simulink model "MATE_SwitchedReluctanceMotor64Drive"  (R2024b)
settings: Solver=FixedStepDiscrete  StartTime=0.0  StopTime=5  FixedStep=Ts  RelTol=1e-3  AbsTol=1e-5  EnableMultiTasking=on
PreLoadFcn:
  | Ts=1e-6;Rsnu=100; Csnu=1e-6;
  | 
  | % Magnetisation characteristic table of the switched Reluctance Motor:
  | % Table elements =  Flux linkage, in Wb.
  | 
  | FluxTable = [
  |     0             0              0             0             0             0
  |     0.3220    0.3050    0.2280    0.1240    0.0220    0.0170
  |     0.3760    0.3570    0.2770    0.1600    0.0420    0.0340
  |     0.3990    0.3850    0.3000    0.1830    0.0640    0.0500
  |     0.4160    0.4020    0.3200    0.2010    0.0840    0.0670
  |     0.4280    0.4150    0.3340    0.2190    0.1030    0.0840
  |     0.4370    0.4260    0.3480    0.2370    0.1230    0.1010
  |     0.4430    0.4330    0.3590    0.2530    0.1420    0.1170
  |     0.4490    0.4390    0.3710    0.2680    0.1610    0.1340
  |     0.4540    0.4440    0.3820    0.2820    0.1790    0.1510
  |     0.4590    0.4490    0.3920    0.2950    0.1970    0.1680
  |     0.4630    0.4530    0.4020    0.3090    0.2140    0.1840
  |     0.4670    0.4570    0.4110    0.3220    0.2310    0.2010
  |     0.4700    0.4620    0.4190    0.3360    0.2460    0.2180
  |     0.4740    0.4650    0.4270    0.3480    0.2610    0.2350
  |     0.4780    0.4690    0.4330    0.3590    0.2770    0.2510
  |     0.4810    0.4730    0.4380    0.3690    0.2910    0.2680
  |     0.4840    0.4770    0.4440    0.3800    0.3050    0.2850
  |     0.4870    0.4790    0.4480    0.3890    0.3200    0.3020];
  | 
  | % Table columns :  Rotor angles, in degrees.
  | 
  | RotorAngles = [
  |     0             10            20            30            40            45];
  | 
  | % Table rows : Stator current, in A.
  | 
  | StatorCurrents = [ 0:size(FluxTable,1)-1] * 25;
PostLoadFcn:
  | Ts=1e-6;Rsnu=100; Csnu=1e-6;
  | 
  | % Magnetisation characteristic table of the switched Reluctance Motor:
  | % Table elements =  Flux linkage, in Wb.
  | 
  | FluxTable = [
  |     0             0              0             0             0             0
  |     0.3220    0.3050    0.2280    0.1240    0.0220    0.0170
  |     0.3760    0.3570    0.2770    0.1600    0.0420    0.0340
  |     0.3990    0.3850    0.3000    0.1830    0.0640    0.0500
  |     0.4160    0.4020    0.3200    0.2010    0.0840    0.0670
  |     0.4280    0.4150    0.3340    0.2190    0.1030    0.0840
  |     0.4370    0.4260    0.3480    0.2370    0.1230    0.1010
  |     0.4430    0.4330    0.3590    0.2530    0.1420    0.1170
  |     0.4490    0.4390    0.3710    0.2680    0.1610    0.1340
  |     0.4540    0.4440    0.3820    0.2820    0.1790    0.1510
  |     0.4590    0.4490    0.3920    0.2950    0.1970    0.1680
  |     0.4630    0.4530    0.4020    0.3090    0.2140    0.1840
  |     0.4670    0.4570    0.4110    0.3220    0.2310    0.2010
  |     0.4700    0.4620    0.4190    0.3360    0.2460    0.2180
  |     0.4740    0.4650    0.4270    0.3480    0.2610    0.2350
  |     0.4780    0.4690    0.4330    0.3590    0.2770    0.2510
  |     0.4810    0.4730    0.4380    0.3690    0.2910    0.2680
  |     0.4840    0.4770    0.4440    0.3800    0.3050    0.2850
  |     0.4870    0.4790    0.4480    0.3890    0.3200    0.3020];
  | 
  | % Table columns :  Rotor angles, in degrees.
  | 
  | RotorAngles = [
  |     0             10            20            30            40            45];
  | 
  | % Table rows : Stator current, in A.
  | 
  | StatorCurrents = [ 0:size(FluxTable,1)-1] * 25;
InitFcn:
  | Ts=1e-6;Rsnu=100; Csnu=1e-6;
  | 
  | % Magnetisation characteristic table of the switched Reluctance Motor:
  | % Table elements =  Flux linkage, in Wb.
  | 
  | FluxTable = [
  |     0             0              0             0             0             0
  |     0.3220    0.3050    0.2280    0.1240    0.0220    0.0170
  |     0.3760    0.3570    0.2770    0.1600    0.0420    0.0340
  |     0.3990    0.3850    0.3000    0.1830    0.0640    0.0500
  |     0.4160    0.4020    0.3200    0.2010    0.0840    0.0670
  |     0.4280    0.4150    0.3340    0.2190    0.1030    0.0840
  |     0.4370    0.4260    0.3480    0.2370    0.1230    0.1010
  |     0.4430    0.4330    0.3590    0.2530    0.1420    0.1170
  |     0.4490    0.4390    0.3710    0.2680    0.1610    0.1340
  |     0.4540    0.4440    0.3820    0.2820    0.1790    0.1510
  |     0.4590    0.4490    0.3920    0.2950    0.1970    0.1680
  |     0.4630    0.4530    0.4020    0.3090    0.2140    0.1840
  |     0.4670    0.4570    0.4110    0.3220    0.2310    0.2010
  |     0.4700    0.4620    0.4190    0.3360    0.2460    0.2180
  |     0.4740    0.4650    0.4270    0.3480    0.2610    0.2350
  |     0.4780    0.4690    0.4330    0.3590    0.2770    0.2510
  |     0.4810    0.4730    0.4380    0.3690    0.2910    0.2680
  |     0.4840    0.4770    0.4440    0.3800    0.3050    0.2850
  |     0.4870    0.4790    0.4480    0.3890    0.3200    0.3020];
  | 
  | % Table columns :  Rotor angles, in degrees.
  | 
  | RotorAngles = [
  |     0             10            20            30            40            45];
  | 
  | % Table rows : Stator current, in A.
  | 
  | StatorCurrents = [ 0:size(FluxTable,1)-1] * 25;
undefined symbols (not defined in the file or in its folder): DiscIntNeverNeededParam
libraries: ee_lib x12, nesl_utility x10, fl_lib x6, simetranss x5
(part 1 of 2)
Description:
  | Copyright 2008-2017 The MathWorks, Inc.
settings Model: ARTEMISmethode_block_infos=$$__separator__$$  ModifiedByFormat=Kyle  Creator=Kyle Diller  LastModifiedBy=Kyle
settings SolverCC: AutoScaleAbsTol=off  AlgebraicLoopSolver=TrustRegion  InsertRTBMode=Auto
settings DataIOCC: LimitDataPoints=on  SaveFormat=Array  SignalLoggingSaveFormat=ModelDataLogs  ReturnWorkspaceOutputs=off  SignalLoggingName=sigsOut
settings OptimizationCC: ExpressionDepthLimit=2147483647  InitFltsAndDblsToZero=on  LifeSpan=inf
settings DebuggingCC: UnderspecifiedInitializationDetection=Classic  MergeDetectMultiDrivingBlocksExec=none  CheckExecutionContextPreStartOutputMsg=on  SignalResolutionControl=TryResolveAllWithWarning  MultiTaskDSMMsg=warning  MultiTaskCondExecSysMsg=none  FcnCallInpInsideContextMsg=warning  UnconnectedInputMsg=warning  UnconnectedOutputMsg=warning  UnconnectedLineMsg=warning  StateNameClashWarn=warning  SFUnexpectedBacktrackingDiag=warning  SFNoUnconditionalDefaultTransitionDiag=warning  SFExecutionAtInitializationDiag=none  ArithmeticOperatorsInVariantConditions=warning
settings HardwareCC: ProdBitPerPointer=32  ProdBitPerSizeT=32  ProdBitPerPtrDiffT=32  ProdLargestAtomicFloat=None  ProdIntDivRoundTo=Undefined  ProdEndianess=Unspecified  ProdWordSize=32  ProdHWDeviceType=32-bit Generic  TargetUnknown=on
settings ModelReferenceCC: EnableRefExpFcnMdlSchedulingChecks=on  PropagateSignalLabelsOutOfModel=off
settings SFSimCC: SimUseLocalCustomCode=off  CustomCodeUndefinedFunction=UseInterfaceOnly
settings RTWCC: RTWUseLocalCustomCode=off  GPUComputeCapability=3.5
settings CodeAppCC: StateflowObjectComments=on
settings GRTTargetCC: TargetLangStandard=C89/C90 (ANSI)  CombineOutputUpdateFcns=off  GRTInterface=on
settings ConfigComp: CovMetricSettings=dw  CovSaveCumulativeToWorkspaceVar=on  CovSaveSingleToWorkspaceVar=on  CovExternalEMLEnable=off  CovSFcnEnable=off
settings SimscapeCC: SimscapeNormalizeSystem=off

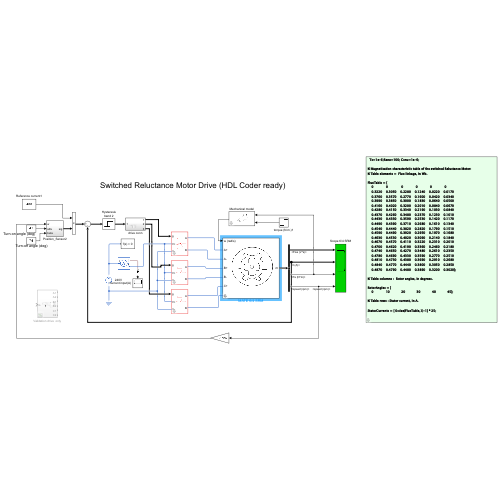
[thumbnail: Simulink's stored preview of the top-level diagram]
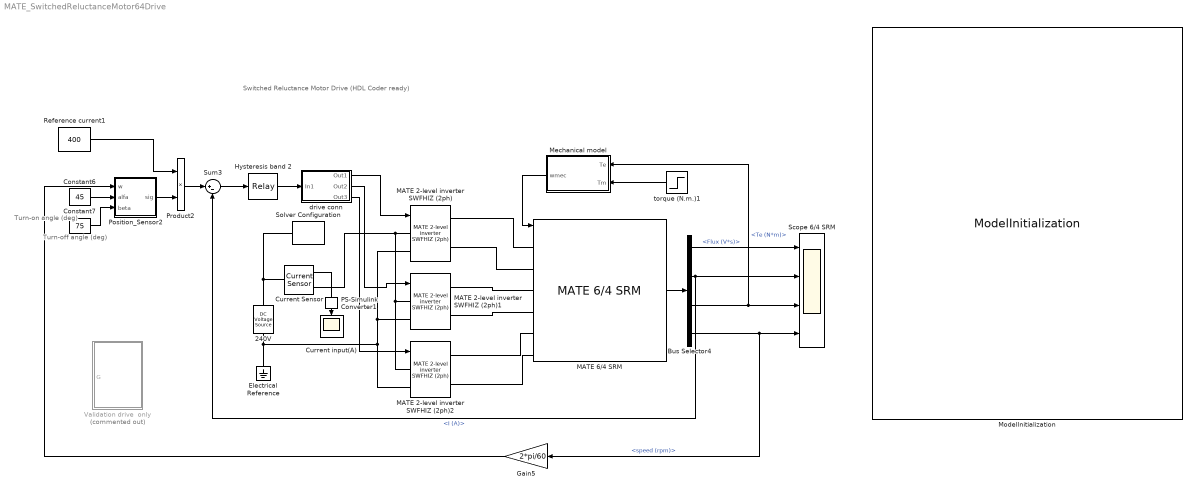
== system MATE_SwitchedReluctanceMotor64Drive ==
  note: Switched Reluctance Motor Drive (HDL Coder ready)
  note: Turn-off angle (deg)
  note: Turn-on angle (deg)
  240V : fl_lib/Electrical/Electrical Sources/DC Voltage Source  v0=240 V
  Bus Selector4 : BusSelector  OutputSignals=Flux (V*s),I (A),Te (N*m),speed (rpm)
  Constant6 : Constant  Value=45
  Constant7 : Constant  Value=75
  Current Sensor : fl_lib/Electrical/Electrical Sensors/Current Sensor
  Current input(A) : Scope
  Electrical Reference : fl_lib/Electrical/Electrical Elements/Electrical Reference
  Gain5 : Gain  Gain=2*pi/60  SaturateOnIntegerOverflow=on  OutDataTypeStr=Inherit: Same as input  ParamDataTypeStr=Inherit: Same as input
  Hysteresis band 2 : Relay  OnSwitchValue=10  OffSwitchValue=-10  SampleTime=Ts
  MATE 2-level inverter SWFHIZ (2ph) : simetranss/FPGA/MATE 2-level inverter SWFHIZ (2ph)  Ron=1e-3  Vf=0.8  Gpp=Rsnu  Gip=Csnu  Ts=Ts  min_charge=0.1
  MATE 2-level inverter SWFHIZ (2ph)1 : simetranss/FPGA/MATE 2-level inverter SWFHIZ (2ph)  Ron=1e-3  Vf=0.8  Gpp=Rsnu  Gip=Csnu  Ts=Ts  min_charge=0.1
  MATE 2-level inverter SWFHIZ (2ph)2 : simetranss/FPGA/MATE 2-level inverter SWFHIZ (2ph)  Ron=1e-3  Vf=0.8  Gpp=Rsnu  Gip=Csnu  Ts=Ts  min_charge=0.1
  MATE 6/4 SRM : simetranss/Machines/MATE 6//4 SRM  MachineType=6/4  Rs=0.05  Inertia=0.05  FluxTable=FluxTable  RotorAngles=RotorAngles  StatorCurrents=StatorCurrents  Friction=0.02  Initialangle=0  TsBlock=-1  nb_points=[100,20,20]  PlotCurves=on
  Mechanical model : Subsystem  mask(Machine rotational mechanical model){J=0.5, F=0.02, fo=0, Ts=Ts}
      mask prompts: J "Inertia (kg.m^2)"; F "Friction (N.m.s)"; fo "Initial mechanical frequency (Hz)"; Ts "Sample Time (s)"
      mask help:
      | This block can implement a simple rotating mechanical equation for machines
      |
      | The block working equation is:
      | wmec=1/J*INT{( Te - Tm -F*wmec )*dt}
      |
      | All values in SI.
      |
      | Parameters:
      | Inertia J (kg.m^2)
      | Friction F (N.m.s)
      | Initial mechanical frequency (Hz)
      | Sample Time (s).
      |
      | Signals:
      | Te: electric torque input from the machine (N.m.)
      | Tm : mechanical torque applied to the shaft (N.m.)
      | wmec: mechanical speed of machine (rad/s)
      |
      | Conversion from Per-Unit values
      |
      | J=2*H*Pn/w_mec^2
      | F=D*Pn/w_mec^2
      | where:
      | J is the inertia in km.m^2
      | H is the inertia constant in seconds.
      | F is the friction factor in N.m.s
      | D in the friction factor or damping factor in pu.
      | Pn is the nominal power of the machine
      | w_mec is the nominal mechanical rotational frequency of the machine in rad/s
  ModelInitialization : simetranss/Usefulls/ModelInitialization  InitFcnX=|  prel=on  posl=on  inif=on  strf=off
      | Ts=1e-6;Rsnu=100; Csnu=1e-6; 
      | 
      | % Magnetisation characteristic table of the switched Reluctance Motor:
      | % Table elements =  Flux linkage, in Wb.
      | 
      | FluxTable = [
      |     0             0              0             0             0             0
      |     0.3220    0.3050    0.2280    0.1240    0.0220    0.0170
      |     0.3760    0.3570    0.2770    0.1600    0.0420    0.0340
      |     0.3990    0.3850    0.3000    0.1830    0.0640    0.0500
      |     0.4160    0.4020    0.3200    0.2010    0.0840    0.0670
      |     0.4280    0.4150    0.3340    0.2190    0.1030    0.0840
      |     0.4370    0.4260    0.3480    0.2370    0.1230    0.1010
      |     0.4430    0.4330    0.3590    0.2530    0.1420    0.1170
      |     0.4490    0.4390    0.3710    0.2680    0.1610    0.1340
      |     0.4540    0.4440    0.3820    0.2820    0.1790    0.1510
      |     0.4590    0.4490    0.3920    0.2950    0.1970    0.1680
      |     0.4630    0.4530    0.4020    0.3090    0.2140    0.1840
      |     0.4670    0.4570    0.4110    0.3220    0.2310    0.2010
      |     0.4700    0.4620    0.4190    0.3360    0.2460    0.2180
      |     0.4740    0.4650    0.4270    0.3480    0.2610    0.2350
      |     0.4780    0.4690    0.4330    0.3590    0.2770    0.2510
      |     0.4810    0.4730    0.4380    0.3690    0.2910    0.2680
      |     0.4840    0.4770    0.4440    0.3800    0.3050    0.2850
      |     0.4870    0.4790    0.4480    0.3890    0.3200    0.3020]; 
      | 
      | % Table columns :  Rotor angles, in degrees.
      | 
      | RotorAngles = [
      |     0             10            20            30            40            45];
      | 
      | % Table rows : Stator current, in A.
      | 
      | StatorCurrents = [ 0:size(FluxTable,1)-1] * 25;
  PS-Simulink Converter1 : nesl_utility/PS-Simulink Converter  PhysicalDomain=network_engine_domain  SubClassName=ps_output  LeftPortType=input  RightPortType=output  PseudoPeriodic=off  Frequencies=[]  VectorFormat=inherit  Unit=inherit  AffineConversion=off
  Position_Sensor2 : Subsystem
  Product2 : Product  SaturateOnIntegerOverflow=on  OutDataTypeStr=Inherit: Same as first input
  Reference current1 : Constant  Value=400
  Scope 6/4 SRM : Scope  NumInputPorts=4
  Solver Configuration : nesl_utility/Solver Configuration  PhysicalDomain=network_engine_domain  SubClassName=solver  LeftPortType=input  RightPortType=generic  Tones=[]  Harmonics=[]  SimulateNoise=off  Profile=off  UseLocalSampling=off  EnableSwitchedLinearOptims=on  FrequencyDomain=off  UseCCode=off  RelTol=0.001  AbsTol=0.001  MinStep=1e-09  ToWorkspace=off  RevertToSquareIcSolve=off  NumHomotopyIterations=100  PhasorMode=off  PhasorModeNumHarmonics=1  ConsistencySolver=NEWTON_XTOL_AFTER_FTOL  IndexReductionMethod=DerivativeReplacement  DoDC=off  ResidualTolerance=1e-09  ConsistencyTolSource=GLOBAL  ConsistencyAbsTol=0.001  ConsistencyRelTol=0.001  ConsistencyTolFactor=0.001  UseLocalSolver=on  LocalSolverChoice=NE_BACKWARD_EULER_ADVANCER  ResolveIndetEquations=on  FunctionEvalNumThread=1  LocalSolverSampleTime=Ts  DoFixedCost=on  MaxNonlinIter=1  MaxModeIter=2  ComputeImpulses=off  ImpulseIterations=2  LinearAlgebra=auto  LinearAlgebraNumThread=0  EquationFormulation=NE_TIME_EF  DelaysMemoryBudget=1024  AutomaticFiltering=on  FilteringTimeConstant=0.001  PartitionStorageMethod=AS_NEEDED  PartitionMemoryBudget=1024  PartitionMethod=ROBUST  MultibodyUseLocalSolver=off  MultibodyLocalSolverChoice=ODE1  MultibodyLocalSolverSampleTime=0.001
  Sum3 : Sum  Inputs=|+-  SaturateOnIntegerOverflow=on
  Validation drive  only : Subsystem  Commented=on
  drive conn : Subsystem
  torque (N.m.)1 : Step  After=100  SampleTime=0
  wires:
  Bus Selector4/3 -> Mechanical model/1(Te), Scope 6/4 SRM/3  "<Te (N*m)>"
  Constant6/1 -> Position_Sensor2/2(alfa)
  Constant7/1 -> Position_Sensor2/3(beta)
  Sum3/1 -> Hysteresis band 2/1
  Product2/1 -> Sum3/1
  Position_Sensor2/1(sig) -> Product2/2
  MATE 6/4 SRM/1 -> Bus Selector4/1
  Bus Selector4/1 -> Scope 6/4 SRM/1  "<Flux (V*s)>"
  Bus Selector4/2 -> Scope 6/4 SRM/2, Sum3/2  "<I (A)>"
  Bus Selector4/4 -> Scope 6/4 SRM/4, Gain5/1  "<speed (rpm)>"
  torque (N.m.)1/1 -> Mechanical model/2(Tm)
  Gain5/1 -> Position_Sensor2/1(w)
  Mechanical model/1(wmec) -> MATE 6/4 SRM/1
  Reference current1/1 -> Product2/1
  PS-Simulink Converter1/1 -> Current input(A)/1
  Hysteresis band 2/1 -> drive conn/1(In1)
  drive conn/1(Out1) -> MATE 2-level inverter SWFHIZ (2ph)/1
  drive conn/2(Out2) -> MATE 2-level inverter SWFHIZ (2ph)1/1
  drive conn/3(Out3) -> MATE 2-level inverter SWFHIZ (2ph)2/1
  connections:
  Solver Configuration/RConn1 -- 240V/LConn1 -- Current Sensor/LConn1
  240V/RConn1 -- Electrical Reference/LConn1 -- MATE 2-level inverter SWFHIZ (2ph)1/LConn2 -- MATE 2-level inverter SWFHIZ (2ph)/LConn2 -- MATE 2-level inverter SWFHIZ (2ph)2/LConn2
  Current Sensor/RConn1 -- PS-Simulink Converter1/LConn1
  Current Sensor/RConn2 -- MATE 2-level inverter SWFHIZ (2ph)2/LConn1 -- MATE 2-level inverter SWFHIZ (2ph)1/LConn1 -- MATE 2-level inverter SWFHIZ (2ph)/LConn1
  MATE 2-level inverter SWFHIZ (2ph)/RConn1 -- MATE 6/4 SRM/LConn1
  MATE 2-level inverter SWFHIZ (2ph)1/RConn2 -- MATE 6/4 SRM/LConn4
  MATE 2-level inverter SWFHIZ (2ph)/RConn2 -- MATE 6/4 SRM/LConn2
  MATE 2-level inverter SWFHIZ (2ph)1/RConn1 -- MATE 6/4 SRM/LConn3
  MATE 2-level inverter SWFHIZ (2ph)2/RConn2 -- MATE 6/4 SRM/LConn6
  MATE 2-level inverter SWFHIZ (2ph)2/RConn1 -- MATE 6/4 SRM/LConn5

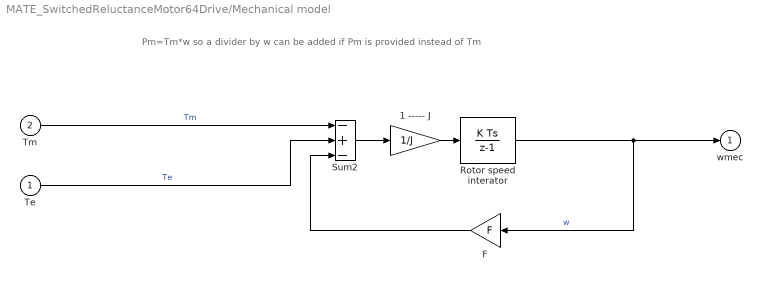
== system MATE_SwitchedReluctanceMotor64Drive/Mechanical model ==
  note: Pm=Tm*w so a divider by w can be added if Pm is provided instead of Tm
  Te : Inport  PortDimensions=1
  Tm : Inport  Port=2
  1 ----- J : Gain  Gain=1/J  SaturateOnIntegerOverflow=on  OutDataTypeStr=Inherit: Same as input  ParamDataTypeStr=Inherit: Same as input
  F : Gain  Gain=F  SaturateOnIntegerOverflow=on  OutDataTypeStr=Inherit: Same as input  ParamDataTypeStr=Inherit: Same as input
  Rotor speed interator : DiscreteIntegrator  InitialCondition=fo*2*pi  SampleTime=Ts  ICPrevOutput=DiscIntNeverNeededParam  ICPrevScaledInput=DiscIntNeverNeededParam
  Sum2 : Sum  Inputs=-+-  InputSameDT=on  SaturateOnIntegerOverflow=on  OutDataTypeStr=Inherit: Same as first input
  wmec : Outport  InitialOutput=0  VectorParamsAs1DForOutWhenUnconnected=off
  wires:
  Tm/1 -> Sum2/1  "Tm"
  Sum2/1 -> 1 ----- J/1
  F/1 -> Sum2/3
  Te/1 -> Sum2/2  "Te"
  1 ----- J/1 -> Rotor speed interator/1
  Rotor speed interator/1 -> wmec/1, F/1  "w"

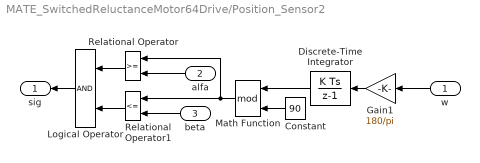
== system MATE_SwitchedReluctanceMotor64Drive/Position_Sensor2 ==
  w : Inport
  alfa : Inport  Port=2
  beta : Inport  Port=3
  Constant : Constant  Value=90
  Discrete-Time Integrator : DiscreteIntegrator  InitialCondition=[0 -30 -60]  SampleTime=Ts  ICPrevOutput=DiscIntNeverNeededParam  ICPrevScaledInput=DiscIntNeverNeededParam
  Gain1 : Gain  Gain=180/pi  SaturateOnIntegerOverflow=on  OutDataTypeStr=Inherit: Same as input  ParamDataTypeStr=Inherit: Same as input
  Logical Operator : Logic  AllPortsSameDT=off
  Math Function : Math  Operator=mod  SignedPower=on
  Relational Operator : RelationalOperator  InputSameDT=off
  Relational Operator1 : RelationalOperator  Operator=<=  InputSameDT=off
  sig : Outport  VectorParamsAs1DForOutWhenUnconnected=off
  wires:
  Logical Operator/1 -> sig/1
  w/1 -> Gain1/1
  Math Function/1 -> Relational Operator/1, Relational Operator1/1
  Relational Operator1/1 -> Logical Operator/2
  Gain1/1 -> Discrete-Time Integrator/1
  beta/1 -> Relational Operator1/2
  alfa/1 -> Relational Operator/2
  Relational Operator/1 -> Logical Operator/1
  Constant/1 -> Math Function/2
  Discrete-Time Integrator/1 -> Math Function/1

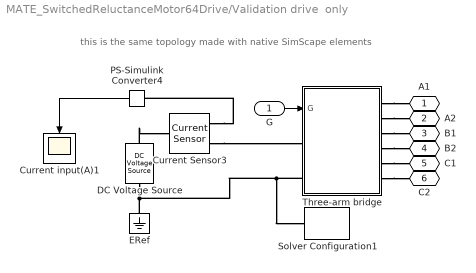
== system MATE_SwitchedReluctanceMotor64Drive/Validation drive  only ==
  note: this is the same topology made with native SimScape elements
  G : Inport
  Current Sensor3 : fl_lib/Electrical/Electrical Sensors/Current Sensor
  Current input(A)1 : Scope
  DC Voltage Source : fl_lib/Electrical/Electrical Sources/DC Voltage Source  v0=240 V
  ERef : fl_lib/Electrical/Electrical Elements/Electrical Reference
  PS-Simulink Converter4 : nesl_utility/PS-Simulink Converter  PhysicalDomain=network_engine_domain  SubClassName=ps_output  LeftPortType=input  RightPortType=output  PseudoPeriodic=off  Frequencies=[]  VectorFormat=inherit  Unit=inherit  AffineConversion=off
  Solver Configuration1 : nesl_utility/Solver Configuration  PhysicalDomain=network_engine_domain  SubClassName=solver  LeftPortType=input  RightPortType=generic  Tones=[]  Harmonics=[]  SimulateNoise=off  Profile=off  UseLocalSampling=off  EnableSwitchedLinearOptims=on  FrequencyDomain=off  UseCCode=off  RelTol=0.001  AbsTol=0.001  MinStep=1e-09  ToWorkspace=off  RevertToSquareIcSolve=off  NumHomotopyIterations=100  PhasorMode=off  PhasorModeNumHarmonics=1  ConsistencySolver=NEWTON_XTOL_AFTER_FTOL  IndexReductionMethod=DerivativeReplacement  DoDC=off  ResidualTolerance=1e-09  ConsistencyTolSource=GLOBAL  ConsistencyAbsTol=0.001  ConsistencyRelTol=0.001  ConsistencyTolFactor=0.001  UseLocalSolver=on  LocalSolverChoice=NE_BACKWARD_EULER_ADVANCER  ResolveIndetEquations=on  FunctionEvalNumThread=1  LocalSolverSampleTime=Ts  DoFixedCost=on  MaxNonlinIter=3  MaxModeIter=2  ComputeImpulses=off  ImpulseIterations=2  LinearAlgebra=auto  LinearAlgebraNumThread=0  EquationFormulation=NE_TIME_EF  DelaysMemoryBudget=1024  AutomaticFiltering=on  FilteringTimeConstant=0.001  PartitionStorageMethod=AS_NEEDED  PartitionMemoryBudget=1024  PartitionMethod=ROBUST  MultibodyUseLocalSolver=off  MultibodyLocalSolverChoice=ODE1  MultibodyLocalSolverSampleTime=0.001
  Three-arm bridge : Subsystem  Tag=PublishSubsystem
  A1 : PMIOPort  Side=Right
  A2 : PMIOPort  Port=2  Side=Right
  B1 : PMIOPort  Port=3  Side=Right
  B2 : PMIOPort  Port=4  Side=Right
  C1 : PMIOPort  Port=5  Side=Right
  C2 : PMIOPort  Port=6  Side=Right
  wires:
  PS-Simulink Converter4/1 -> Current input(A)1/1
  G/1 -> Three-arm bridge/1(G)
  connections:
  Three-arm bridge/LConn2 -- Solver Configuration1/RConn1 -- ERef/LConn1 -- DC Voltage Source/RConn1
  Current Sensor3/RConn2 -- Three-arm bridge/LConn1
  Three-arm bridge/RConn1 -- A1/RConn1
  Current Sensor3/RConn1 -- PS-Simulink Converter4/LConn1
  DC Voltage Source/LConn1 -- Current Sensor3/LConn1
  Three-arm bridge/RConn2 -- A2/RConn1
  Three-arm bridge/RConn3 -- B1/RConn1
  Three-arm bridge/RConn6 -- C2/RConn1
  Three-arm bridge/RConn4 -- B2/RConn1
  Three-arm bridge/RConn5 -- C1/RConn1

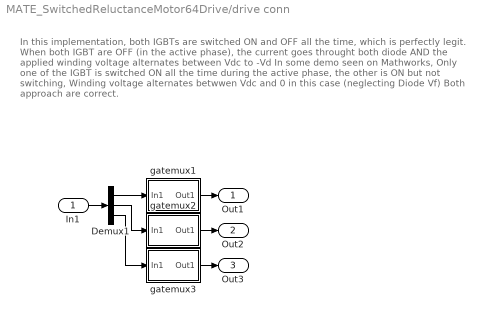
== system MATE_SwitchedReluctanceMotor64Drive/drive conn ==
  note: In this implementation, both IGBTs are switched ON and OFF all the time, which is perfectly legit. When both IGBT are OFF (in the active phase), the current goes throught both diode AND the applied winding voltage alternates between Vdc to -Vd
      |
      | In some demo seen on Mathworks, Only one of the IGBT is switched ON all the time during the active phase, the other is ON but not switching, Winding voltage alternates betwwen Vdc and 0 in this case (neglecting Diode Vf)
      |
      | Both approach are correct.
  In1 : Inport
  Demux1 : Demux  Outputs=3
  gatemux1 : Subsystem
  gatemux2 : Subsystem
  gatemux3 : Subsystem
  Out1 : Outport
  Out2 : Outport  Port=2
  Out3 : Outport  Port=3
  wires:
  Demux1/2 -> gatemux2/1(In1)
  gatemux1/1(Out1) -> Out1/1
  Demux1/1 -> gatemux1/1(In1)
  Demux1/3 -> gatemux3/1(In1)
  gatemux2/1(Out1) -> Out2/1
  gatemux3/1(Out1) -> Out3/1
  In1/1 -> Demux1/1

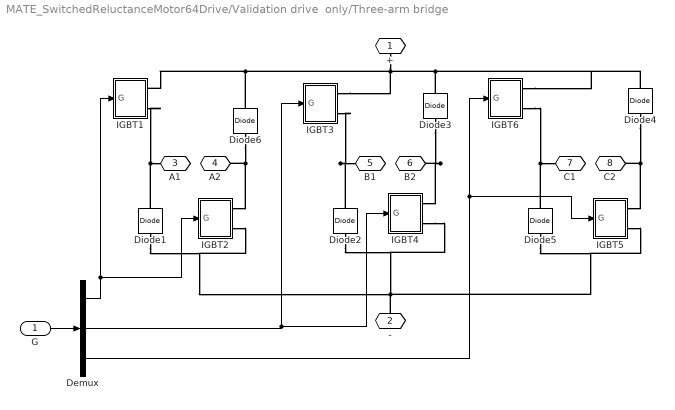
== system MATE_SwitchedReluctanceMotor64Drive/Validation drive  only/Three-arm bridge ==
  G : Inport
  Demux : Demux  Outputs=3
  Diode{1..6} (6 alike) : ee_lib/Semiconductors & Converters/Diode  ModelType=ee.enum.diode.modelType.pwl  TableType=ee.enum.diode.tableType.IfMat  IfMat=[.07, .12, .19, 1.75, 4.24, 7.32, 11.2; .16, .3, .72, 2.14, 5.02, 8.35, 13.12] A  VfMat=[.9, 1.15, 1.25, 1.5, 1.75, 2.17, 2.6, 2.85; .58, .68, .75, 1.1, 1.38, 1.77, 2.27, 2.7] V  TjVec=[25, 125] degC  VfVec=[.5, .7, .9, 1.3, 1.7, 2.1, 2.5] V  IfVec=[.1, .2, .5, 1, 2, 4, 7, 10] A  IrMat=[1e-06, 2e-06, 5e-06, 1e-05, 2.5e-05, 5e-05, .0001; 2e-06, 5e-06, 1e-05, 4e-05, 8e-05, .0002, .0005] A  VrMat=[10, 100, 200, 250, 300, 325, 350; 10, 70, 160, 220, 270, 300, 320] V  VrVec=[10, 20, 40, 50, 70, 80, 100] V  IrVec=[1e-06, 2e-06, 5e-06, 1e-05, 2e-05, 5e-05, .0001] A  Vf=0.1 V  Ron=0.01 Ohm  Goff=1e-8 1/Ohm  prmExp=ee.enum.diode.expParam.useTwo  I12=[.0137, .545] A  V12=[.6, .7] V  RS=0 Ohm  Tmeas=25 degC  IS=1e-12 A  ec=1  I1=0.0137 A  V1=0.6 V  N_series=1  N_parallel=1  ZenerEnable=false  Rz=0.3 Ohm  BV=inf V  C_param=ee.enum.diode.capParam.fixed  CJ=0 pF  CJ0=5 pF  Vvec=[.1, 10, 100] V  Cvec=[3.5, 1, .4] pF  VJ=1 V  Mgrad=0.5  FC=0.5  Q_param=ee.enum.diode.recoveryParam.off  iRM=-7.15 A  iF=4 A  didt=-750 A/us  trr_factor=3  trr=115 ns  Qrr=150 s*nA  Vr=-600 V  Ls=150 nH  Erec=0.03 J  TT=50 ns  tau=100 ns  T_param=ee.enum.diode.temperatureParam.off  Tdevice=25 degC  I1_T2=0.245 A  V1_T2=0.5 V  IS_T2=1.25e-7 A  Tmeas2=125 degC  XTI_param=ee.enum.diode.xtiParam.pn  XTI=3  EG_param=ee.enum.diode.egapParam.material_si  EG=1.11 eV  dBVdT=0 V/K  fault_action=simscape.enum.assert.action.none  t_fault=inf s  enable_fault_input=simscape.enum.onoff.off  i_specify=off  i_priority=None  i=0 A  i_nominal_specify=off  i_nominal_value=1  i_nominal_unit=A  v_specify=off  v_priority=None  v=0 V  v_nominal_specify=off  v_nominal_value=1  v_nominal_unit=V  v_capacitor_specify=off  v_capacitor_priority=None  v_capacitor=0 V  v_capacitor_nominal_specify=off  v_capacitor_nominal_value=1  v_capacitor_nominal_unit=V  Qj_specify=off  Qj_priority=High  Qj=0 C  Qj_nominal_specify=off  Qj_nominal_value=1  Qj_nominal_unit=C  i_diode_specify=off  i_diode_priority=None  i_diode=0 A  i_diode_nominal_specify=off  i_diode_nominal_value=1  i_diode_nominal_unit=A  v_diode_specify=off  v_diode_priority=None  v_diode=0 V  v_diode_nominal_specify=off  v_diode_nominal_value=1  v_diode_nominal_unit=V  i_capacitor_specify=off  i_capacitor_priority=None  i_capacitor=0 A  i_capacitor_nominal_specify=off  i_capacitor_nominal_value=1  i_capacitor_nominal_unit=A  power_dissipated_specify=off  power_dissipated_priority=None  power_dissipated=0 W  power_dissipated_nominal_specify=off  power_dissipated_nominal_value=1  power_dissipated_nominal_unit=W  fidelity_level=ee.enum.diode.fidelity.includeChargeDyn  rec_loss_model=ee.enum.diode.reverseRecoveryModel.fixed  ErecVal=0 J  scaleWithIandV=true  ErecMat=zeros(2, 3) J  TjrecVec=[298.15, 398.15] K  IfrecVec=[.1, 1, 10] A  IrecVal=10 A  VrecVal=10 V  tFilter=1 / 1000 / 100 s  thermal_network_parameterization=ee.enum.thermalNetworkTopology.junctionCase  Rth=[0, 10] K/W  Rth_Cauer=[1, 3, 10] K/W  Rth_Foster=[4, 6] K/W  thermal_mass_parameterization=ee.enum.thermalNetwork.timeconstant  thermal_mass=[0, 1] J/K  thermal_mass_Cauer=[.1, .3, 1] J/K  thermal_mass_Foster=[1.5, 3] J/K  thermal_time_constant=[0, 10] s  thermal_time_constant_Cauer=[1, 3, 10] s  thermal_time_constant_Foster=[6, 18] s  thermal_mass_initial_temperatures=[25, 25] degC  thermal_mass_initial_temperatures_Cauer=[25, 25, 25] degC  junction_thermal_mass=0.01 J/K  Tvec_initial_Foster=[25, 25, 25, 25] degC  no_thermal_network=0  junction_temperature_specify=off  junction_temperature_priority=None  junction_temperature=25 degC  junction_temperature_nominal_specify=off  junction_temperature_nominal_value=1  junction_temperature_nominal_unit=degC
  IGBT1 : Subsystem
  IGBT2 : Subsystem
  IGBT3 : Subsystem
  IGBT4 : Subsystem
  IGBT5 : Subsystem
  IGBT6 : Subsystem
  + : PMIOPort  Side=Left
  - : PMIOPort  Port=2  Side=Left
  A1 : PMIOPort  Port=3  Side=Right
  A2 : PMIOPort  Port=4  Side=Right
  B1 : PMIOPort  Port=5  Side=Right
  B2 : PMIOPort  Port=6  Side=Right
  C1 : PMIOPort  Port=7  Side=Right
  C2 : PMIOPort  Port=8  Side=Right
  wires:
  Demux/1 -> IGBT2/1(G), IGBT1/1(G)
  G/1 -> Demux/1
  Demux/2 -> IGBT4/1(G), IGBT3/1(G)
  Demux/3 -> IGBT5/1(G), IGBT6/1(G)
  connections:
  IGBT1/RConn2 -- A1/RConn1 -- Diode1/RConn1
  IGBT4/RConn2 -- Diode2/LConn1 -- -/RConn1 -- IGBT2/RConn2 -- Diode1/LConn1 -- IGBT5/RConn2 -- Diode5/LConn1
  Diode3/RConn1 -- IGBT6/RConn1 -- Diode4/RConn1 -- IGBT3/RConn1 -- Diode6/RConn1 -- IGBT1/RConn1 -- +/RConn1
  C1/RConn1 -- IGBT6/RConn2 -- Diode5/RConn1
  B1/RConn1 -- IGBT3/RConn2 -- Diode2/RConn1
  A2/RConn1 -- IGBT2/RConn1 -- Diode6/LConn1
  B2/RConn1 -- IGBT4/RConn1 -- Diode3/LConn1
  C2/RConn1 -- IGBT5/RConn1 -- Diode4/LConn1

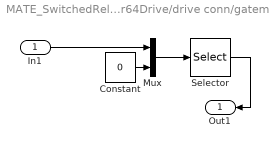
== system MATE_SwitchedReluctanceMotor64Drive/drive conn/gatemux1 ==
  In1 : Inport
  Constant : Constant  Value=0
  Mux : Mux  Inputs=2
  Selector : Selector  InputPortWidth=2  IndexOptions=Index vector (dialog)  Indices=[1 2 2 1]  OutputSizes=1
  Out1 : Outport
  wires:
  Selector/1 -> Out1/1
  In1/1 -> Mux/1
  Mux/1 -> Selector/1
  Constant/1 -> Mux/2

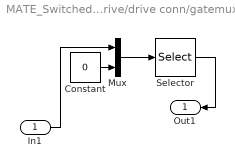
== system MATE_SwitchedReluctanceMotor64Drive/drive conn/gatemux2 ==
  In1 : Inport
  Constant : Constant  Value=0
  Mux : Mux  Inputs=2
  Selector : Selector  InputPortWidth=2  IndexOptions=Index vector (dialog)  Indices=[1 2 2 1]  OutputSizes=1
  Out1 : Outport
  wires:
  Constant/1 -> Mux/2
  Mux/1 -> Selector/1
  In1/1 -> Mux/1
  Selector/1 -> Out1/1

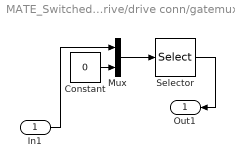
== system MATE_SwitchedReluctanceMotor64Drive/drive conn/gatemux3 ==
  In1 : Inport
  Constant : Constant  Value=0
  Mux : Mux  Inputs=2
  Selector : Selector  InputPortWidth=2  IndexOptions=Index vector (dialog)  Indices=[1 2 2 1]  OutputSizes=1
  Out1 : Outport
  wires:
  Selector/1 -> Out1/1
  In1/1 -> Mux/1
  Mux/1 -> Selector/1
  Constant/1 -> Mux/2

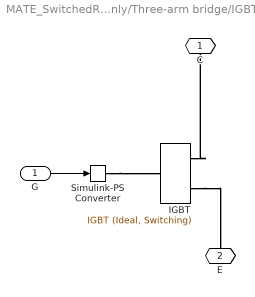
== system MATE_SwitchedReluctanceMotor64Drive/Validation drive  only/Three-arm bridge/IGBT1 ==
  G : Inport
  IGBT : ee_lib/Semiconductors & Converters/IGBT (Ideal, Switching)  port_option=ee.enum.controlport.ps  Vf=0.1 V  Ron=0.01 Ohm  Goff=1e-5 1/Ohm  Vth=0.5 V  diode_param=ee.enum.semiconductors.protectionDiode.external  diode_Vf=0.6 V  diode_Ron=0.03 Ohm  diode_Goff=1e-5 1/Ohm  diode_C=5e-8 F  diode_iRM=-235 A  diode_iF=300 A  diode_idot=-50 A/us  diode_trr_param=1  diode_trr_factor=3  diode_trr=15 us  diode_Qrr=1.5e+3 s*uA  ice_specify=off  ice_priority=None  ice=0 A  ice_nominal_specify=off  ice_nominal_value=1  ice_nominal_unit=A  vce_specify=off  vce_priority=None  vce=0 V  vce_nominal_specify=off  vce_nominal_value=1  vce_nominal_unit=V  vge_specify=off  vge_priority=None  vge=0 V  vge_nominal_specify=off  vge_nominal_value=1  vge_nominal_unit=V  thermal_loss_option=ee.enum.converters.thermalLossOption.constantvalues  Von_data=[0, .1, .6, .8, 1, 1.3, 1.6, 2, 2.4; 0, .1, .7, 1, 1.2, 1.5, 1.9, 2.4, 2.8] V  Tj=[298.15, 398.15] K  Iout_data=[0, .1, 1, 5, 10, 20, 40, 70, 100] A  Eon_data=[0, .0024, .024, .12, .2, .48, 1.04, 2.16, 3.24; 0, .003, .03, .15, .25, .6, 1.3, 2.7, 4.05] * 1e-3 J  Eoff_data=[0, .0007, .0066, .033, .066, .17, .33, .83, 1.5; 0, .001, .01, .05, .1, .25, .5, 1.2, 2.2] * 1e-3 J  Eon_data_3D=[zeros(2, 9, 3)] J  Eoff_data_3D=[zeros(2, 9, 3)] J  Tj_loss=[298.15, 398.15] K  Iout_data_loss=[0, .1, 1, 5, 10, 20, 40, 70, 100] A  tabulateWithVce=false  Vce_loss=[0, 150, 300] V  Eon_scalar=22.86e-3 J  Eoff_scalar=17.14e-3 J  Voff=300 V  Iout_scalar=600 A  useCurrentFromPreviousCycle=false  useVoltageFromPreviousCycle=false  diodeModelType=ee.enum.converters.diodeModelType.pwl  diodeTableType=ee.enum.diode.tableType.IfMat  diode_ReverseIVType=ee.enum.diode.diodeReverseIV.constant  diode_IfMat=[.07, .12, .19, 1.75, 4.24, 7.32, 11.2; .16, .3, .72, 2.14, 4.02, 6.35, 9.12] A  diode_VfMat=[.9, 1.15, 1.25, 1.5, 1.75, 2.17, 2.6, 2.85; .58, .68, .75, 1.1, 1.38, 1.77, 2.27, 2.7] V  diode_TjVec=[25, 125] degC  diode_VfVec=[.5, .7, .9, 1.3, 1.7, 2.1, 2.5] V  diode_IfVec=[.1, .2, .5, 1, 2, 4, 7, 10] A  diode_IrMat=[1e-06, 2e-06, 5e-06, 1e-05, 2.5e-05, 5e-05, .0001; 2e-06, 5e-06, 1e-05, 4e-05, 8e-05, .0002, .0005] A  diode_VrMat=[10, 100, 200, 250, 300, 325, 350; 10, 70, 160, 220, 270, 300, 320] V  diode_VrVec=[10, 20, 40, 50, 70, 80, 100] V  diode_IrVec=[1e-06, 2e-06, 5e-06, 1e-05, 2e-05, 5e-05, .0001] A  diode_Vr=-600 V  diode_Ls=150 nH  diode_Erec=0.03 J  diode_rec_loss_model=ee.enum.diode.reverseRecoveryModel.fixed  diode_ErecVal=0 J  diode_scaleWithIandV=true  diode_ErecMat=zeros(2, 3) J  diode_TjrecVec=[298.15, 398.15] K  diode_IfrecVec=[.1, 1, 10] A  diode_IrecVal=10 A  diode_VrecVal=10 V  diode_tFilter=1 / 1000 / 100 s  separateThermalPortForDiode=false  thermal_network_parameterization=ee.enum.thermalNetworkTopology.external  Rth=[.08, .5] K/W  Rth_Cauer=[.08, .1, .5] K/W  Rth_Foster=[.08, .14, .22, .16] K/W  thermal_mass_parameterization=ee.enum.thermalNetwork.timeconstant  thermal_mass=[.01, .5] J/K  thermal_mass_Cauer=[.01, .1, .5] J/K  thermal_mass_Foster=[.001, .005, .05, .5] J/K  thermal_time_constant=[.001, .2] s  thermal_time_constant_Cauer=[.001, .1, .2] s  thermal_time_constant_Foster=[7e-05, .0007, .01, .08] s  thermal_mass_initial_temperatures=[25, 25] degC  thermal_mass_initial_temperatures_Cauer=[25, 25, 25] degC  junction_thermal_mass=0.01 J/K  Tvec_initial_Foster=[25, 25, 25, 25] degC  RthDiode=[.03, .2] K/W  RthCauerDiode=[.03, .1, .2] K/W  RthFosterDiode=[.03, .2] K/W  thermalMassDiode=[3, 25] J/K  thermalMassCauerDiode=[3, 10, 25] J/K  thermalMassFosterDiode=[33, 50] J/K  thermalTauDiode=[.1, 5] s  thermalTauCauerDiode=[.1, 1, 5] s  thermalTauFosterDiode=[1, 10] s  thermalMassInitTempDiode=[25, 25] degC  thermalMassInitTempCauerDiode=[25, 25, 25] degC  junctionthermalMassDiode=0.1 J/K  TVecInitialFosterDiode=[25, 25, 25, 25] degC  no_thermal_network=0  IGBT_junction_temperature_specify=off  IGBT_junction_temperature_priority=None  IGBT_junction_temperature=25 degC  IGBT_junction_temperature_nominal_specify=off  IGBT_junction_temperature_nominal_value=1  IGBT_junction_temperature_nominal_unit=degC  diode_junction_temperature_specify=off  diode_junction_temperature_priority=None  diode_junction_temperature=25 degC  diode_junction_temperature_nominal_specify=off  diode_junction_temperature_nominal_value=1  diode_junction_temperature_nominal_unit=degC  Qj_specify=off  Qj_priority=None  Qj=0 W  Qj_nominal_specify=off  Qj_nominal_value=1  Qj_nominal_unit=W  accumulatedSwitchingLosses_specify=off  accumulatedSwitchingLosses_priority=None  accumulatedSwitchingLosses=0 J
  Simulink-PS Converter : nesl_utility/Simulink-PS Converter  PhysicalDomain=network_engine_domain  SubClassName=ps_input  LeftPortType=input  RightPortType=output  PseudoPeriodic=off  Frequencies=[]  NoiseDistribution=none  NoiseParameters=[]  Unit=V  AffineConversion=off  FilteringAndDerivatives=zero  SimscapeFilterOrder=1  InputFilterTimeConstant=.001  UdotUserProvided=1
  C : PMIOPort  Side=Right
  E : PMIOPort  Port=2  Side=Right
  wires:
  G/1 -> Simulink-PS Converter/1
  connections:
  IGBT/RConn1 -- C/RConn1
  IGBT/RConn2 -- E/RConn1
  Simulink-PS Converter/RConn1 -- IGBT/LConn1

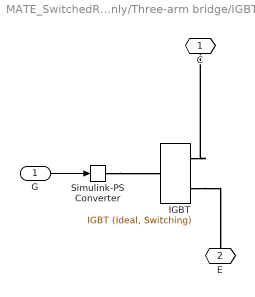
== system MATE_SwitchedReluctanceMotor64Drive/Validation drive  only/Three-arm bridge/IGBT2 ==
  G : Inport
  IGBT : ee_lib/Semiconductors & Converters/IGBT (Ideal, Switching)  port_option=ee.enum.controlport.ps  Vf=0.1 V  Ron=0.01 Ohm  Goff=1e-5 1/Ohm  Vth=0.5 V  diode_param=ee.enum.semiconductors.protectionDiode.external  diode_Vf=0.6 V  diode_Ron=0.03 Ohm  diode_Goff=1e-5 1/Ohm  diode_C=5e-8 F  diode_iRM=-235 A  diode_iF=300 A  diode_idot=-50 A/us  diode_trr_param=1  diode_trr_factor=3  diode_trr=15 us  diode_Qrr=1.5e+3 s*uA  ice_specify=off  ice_priority=None  ice=0 A  ice_nominal_specify=off  ice_nominal_value=1  ice_nominal_unit=A  vce_specify=off  vce_priority=None  vce=0 V  vce_nominal_specify=off  vce_nominal_value=1  vce_nominal_unit=V  vge_specify=off  vge_priority=None  vge=0 V  vge_nominal_specify=off  vge_nominal_value=1  vge_nominal_unit=V  thermal_loss_option=ee.enum.converters.thermalLossOption.constantvalues  Von_data=[0, .1, .6, .8, 1, 1.3, 1.6, 2, 2.4; 0, .1, .7, 1, 1.2, 1.5, 1.9, 2.4, 2.8] V  Tj=[298.15, 398.15] K  Iout_data=[0, .1, 1, 5, 10, 20, 40, 70, 100] A  Eon_data=[0, .0024, .024, .12, .2, .48, 1.04, 2.16, 3.24; 0, .003, .03, .15, .25, .6, 1.3, 2.7, 4.05] * 1e-3 J  Eoff_data=[0, .0007, .0066, .033, .066, .17, .33, .83, 1.5; 0, .001, .01, .05, .1, .25, .5, 1.2, 2.2] * 1e-3 J  Eon_data_3D=[zeros(2, 9, 3)] J  Eoff_data_3D=[zeros(2, 9, 3)] J  Tj_loss=[298.15, 398.15] K  Iout_data_loss=[0, .1, 1, 5, 10, 20, 40, 70, 100] A  tabulateWithVce=false  Vce_loss=[0, 150, 300] V  Eon_scalar=22.86e-3 J  Eoff_scalar=17.14e-3 J  Voff=300 V  Iout_scalar=600 A  useCurrentFromPreviousCycle=false  useVoltageFromPreviousCycle=false  diodeModelType=ee.enum.converters.diodeModelType.pwl  diodeTableType=ee.enum.diode.tableType.IfMat  diode_ReverseIVType=ee.enum.diode.diodeReverseIV.constant  diode_IfMat=[.07, .12, .19, 1.75, 4.24, 7.32, 11.2; .16, .3, .72, 2.14, 4.02, 6.35, 9.12] A  diode_VfMat=[.9, 1.15, 1.25, 1.5, 1.75, 2.17, 2.6, 2.85; .58, .68, .75, 1.1, 1.38, 1.77, 2.27, 2.7] V  diode_TjVec=[25, 125] degC  diode_VfVec=[.5, .7, .9, 1.3, 1.7, 2.1, 2.5] V  diode_IfVec=[.1, .2, .5, 1, 2, 4, 7, 10] A  diode_IrMat=[1e-06, 2e-06, 5e-06, 1e-05, 2.5e-05, 5e-05, .0001; 2e-06, 5e-06, 1e-05, 4e-05, 8e-05, .0002, .0005] A  diode_VrMat=[10, 100, 200, 250, 300, 325, 350; 10, 70, 160, 220, 270, 300, 320] V  diode_VrVec=[10, 20, 40, 50, 70, 80, 100] V  diode_IrVec=[1e-06, 2e-06, 5e-06, 1e-05, 2e-05, 5e-05, .0001] A  diode_Vr=-600 V  diode_Ls=150 nH  diode_Erec=0.03 J  diode_rec_loss_model=ee.enum.diode.reverseRecoveryModel.fixed  diode_ErecVal=0 J  diode_scaleWithIandV=true  diode_ErecMat=zeros(2, 3) J  diode_TjrecVec=[298.15, 398.15] K  diode_IfrecVec=[.1, 1, 10] A  diode_IrecVal=10 A  diode_VrecVal=10 V  diode_tFilter=1 / 1000 / 100 s  separateThermalPortForDiode=false  thermal_network_parameterization=ee.enum.thermalNetworkTopology.external  Rth=[.08, .5] K/W  Rth_Cauer=[.08, .1, .5] K/W  Rth_Foster=[.08, .14, .22, .16] K/W  thermal_mass_parameterization=ee.enum.thermalNetwork.timeconstant  thermal_mass=[.01, .5] J/K  thermal_mass_Cauer=[.01, .1, .5] J/K  thermal_mass_Foster=[.001, .005, .05, .5] J/K  thermal_time_constant=[.001, .2] s  thermal_time_constant_Cauer=[.001, .1, .2] s  thermal_time_constant_Foster=[7e-05, .0007, .01, .08] s  thermal_mass_initial_temperatures=[25, 25] degC  thermal_mass_initial_temperatures_Cauer=[25, 25, 25] degC  junction_thermal_mass=0.01 J/K  Tvec_initial_Foster=[25, 25, 25, 25] degC  RthDiode=[.03, .2] K/W  RthCauerDiode=[.03, .1, .2] K/W  RthFosterDiode=[.03, .2] K/W  thermalMassDiode=[3, 25] J/K  thermalMassCauerDiode=[3, 10, 25] J/K  thermalMassFosterDiode=[33, 50] J/K  thermalTauDiode=[.1, 5] s  thermalTauCauerDiode=[.1, 1, 5] s  thermalTauFosterDiode=[1, 10] s  thermalMassInitTempDiode=[25, 25] degC  thermalMassInitTempCauerDiode=[25, 25, 25] degC  junctionthermalMassDiode=0.1 J/K  TVecInitialFosterDiode=[25, 25, 25, 25] degC  no_thermal_network=0  IGBT_junction_temperature_specify=off  IGBT_junction_temperature_priority=None  IGBT_junction_temperature=25 degC  IGBT_junction_temperature_nominal_specify=off  IGBT_junction_temperature_nominal_value=1  IGBT_junction_temperature_nominal_unit=degC  diode_junction_temperature_specify=off  diode_junction_temperature_priority=None  diode_junction_temperature=25 degC  diode_junction_temperature_nominal_specify=off  diode_junction_temperature_nominal_value=1  diode_junction_temperature_nominal_unit=degC  Qj_specify=off  Qj_priority=None  Qj=0 W  Qj_nominal_specify=off  Qj_nominal_value=1  Qj_nominal_unit=W  accumulatedSwitchingLosses_specify=off  accumulatedSwitchingLosses_priority=None  accumulatedSwitchingLosses=0 J
  Simulink-PS Converter : nesl_utility/Simulink-PS Converter  PhysicalDomain=network_engine_domain  SubClassName=ps_input  LeftPortType=input  RightPortType=output  PseudoPeriodic=off  Frequencies=[]  NoiseDistribution=none  NoiseParameters=[]  Unit=V  AffineConversion=off  FilteringAndDerivatives=zero  SimscapeFilterOrder=1  InputFilterTimeConstant=.001  UdotUserProvided=1
  C : PMIOPort  Side=Right
  E : PMIOPort  Port=2  Side=Right
  wires:
  G/1 -> Simulink-PS Converter/1
  connections:
  Simulink-PS Converter/RConn1 -- IGBT/LConn1
  IGBT/RConn2 -- E/RConn1
  IGBT/RConn1 -- C/RConn1

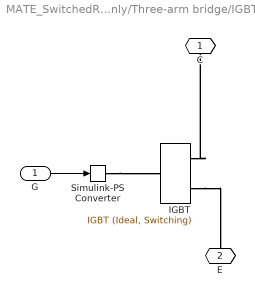
== system MATE_SwitchedReluctanceMotor64Drive/Validation drive  only/Three-arm bridge/IGBT3 ==
  G : Inport
  IGBT : ee_lib/Semiconductors & Converters/IGBT (Ideal, Switching)  port_option=ee.enum.controlport.ps  Vf=0.1 V  Ron=0.01 Ohm  Goff=1e-5 1/Ohm  Vth=0.5 V  diode_param=ee.enum.semiconductors.protectionDiode.external  diode_Vf=0.6 V  diode_Ron=0.03 Ohm  diode_Goff=1e-5 1/Ohm  diode_C=5e-8 F  diode_iRM=-235 A  diode_iF=300 A  diode_idot=-50 A/us  diode_trr_param=1  diode_trr_factor=3  diode_trr=15 us  diode_Qrr=1.5e+3 s*uA  ice_specify=off  ice_priority=None  ice=0 A  ice_nominal_specify=off  ice_nominal_value=1  ice_nominal_unit=A  vce_specify=off  vce_priority=None  vce=0 V  vce_nominal_specify=off  vce_nominal_value=1  vce_nominal_unit=V  vge_specify=off  vge_priority=None  vge=0 V  vge_nominal_specify=off  vge_nominal_value=1  vge_nominal_unit=V  thermal_loss_option=ee.enum.converters.thermalLossOption.constantvalues  Von_data=[0, .1, .6, .8, 1, 1.3, 1.6, 2, 2.4; 0, .1, .7, 1, 1.2, 1.5, 1.9, 2.4, 2.8] V  Tj=[298.15, 398.15] K  Iout_data=[0, .1, 1, 5, 10, 20, 40, 70, 100] A  Eon_data=[0, .0024, .024, .12, .2, .48, 1.04, 2.16, 3.24; 0, .003, .03, .15, .25, .6, 1.3, 2.7, 4.05] * 1e-3 J  Eoff_data=[0, .0007, .0066, .033, .066, .17, .33, .83, 1.5; 0, .001, .01, .05, .1, .25, .5, 1.2, 2.2] * 1e-3 J  Eon_data_3D=[zeros(2, 9, 3)] J  Eoff_data_3D=[zeros(2, 9, 3)] J  Tj_loss=[298.15, 398.15] K  Iout_data_loss=[0, .1, 1, 5, 10, 20, 40, 70, 100] A  tabulateWithVce=false  Vce_loss=[0, 150, 300] V  Eon_scalar=22.86e-3 J  Eoff_scalar=17.14e-3 J  Voff=300 V  Iout_scalar=600 A  useCurrentFromPreviousCycle=false  useVoltageFromPreviousCycle=false  diodeModelType=ee.enum.converters.diodeModelType.pwl  diodeTableType=ee.enum.diode.tableType.IfMat  diode_ReverseIVType=ee.enum.diode.diodeReverseIV.constant  diode_IfMat=[.07, .12, .19, 1.75, 4.24, 7.32, 11.2; .16, .3, .72, 2.14, 4.02, 6.35, 9.12] A  diode_VfMat=[.9, 1.15, 1.25, 1.5, 1.75, 2.17, 2.6, 2.85; .58, .68, .75, 1.1, 1.38, 1.77, 2.27, 2.7] V  diode_TjVec=[25, 125] degC  diode_VfVec=[.5, .7, .9, 1.3, 1.7, 2.1, 2.5] V  diode_IfVec=[.1, .2, .5, 1, 2, 4, 7, 10] A  diode_IrMat=[1e-06, 2e-06, 5e-06, 1e-05, 2.5e-05, 5e-05, .0001; 2e-06, 5e-06, 1e-05, 4e-05, 8e-05, .0002, .0005] A  diode_VrMat=[10, 100, 200, 250, 300, 325, 350; 10, 70, 160, 220, 270, 300, 320] V  diode_VrVec=[10, 20, 40, 50, 70, 80, 100] V  diode_IrVec=[1e-06, 2e-06, 5e-06, 1e-05, 2e-05, 5e-05, .0001] A  diode_Vr=-600 V  diode_Ls=150 nH  diode_Erec=0.03 J  diode_rec_loss_model=ee.enum.diode.reverseRecoveryModel.fixed  diode_ErecVal=0 J  diode_scaleWithIandV=true  diode_ErecMat=zeros(2, 3) J  diode_TjrecVec=[298.15, 398.15] K  diode_IfrecVec=[.1, 1, 10] A  diode_IrecVal=10 A  diode_VrecVal=10 V  diode_tFilter=1 / 1000 / 100 s  separateThermalPortForDiode=false  thermal_network_parameterization=ee.enum.thermalNetworkTopology.external  Rth=[.08, .5] K/W  Rth_Cauer=[.08, .1, .5] K/W  Rth_Foster=[.08, .14, .22, .16] K/W  thermal_mass_parameterization=ee.enum.thermalNetwork.timeconstant  thermal_mass=[.01, .5] J/K  thermal_mass_Cauer=[.01, .1, .5] J/K  thermal_mass_Foster=[.001, .005, .05, .5] J/K  thermal_time_constant=[.001, .2] s  thermal_time_constant_Cauer=[.001, .1, .2] s  thermal_time_constant_Foster=[7e-05, .0007, .01, .08] s  thermal_mass_initial_temperatures=[25, 25] degC  thermal_mass_initial_temperatures_Cauer=[25, 25, 25] degC  junction_thermal_mass=0.01 J/K  Tvec_initial_Foster=[25, 25, 25, 25] degC  RthDiode=[.03, .2] K/W  RthCauerDiode=[.03, .1, .2] K/W  RthFosterDiode=[.03, .2] K/W  thermalMassDiode=[3, 25] J/K  thermalMassCauerDiode=[3, 10, 25] J/K  thermalMassFosterDiode=[33, 50] J/K  thermalTauDiode=[.1, 5] s  thermalTauCauerDiode=[.1, 1, 5] s  thermalTauFosterDiode=[1, 10] s  thermalMassInitTempDiode=[25, 25] degC  thermalMassInitTempCauerDiode=[25, 25, 25] degC  junctionthermalMassDiode=0.1 J/K  TVecInitialFosterDiode=[25, 25, 25, 25] degC  no_thermal_network=0  IGBT_junction_temperature_specify=off  IGBT_junction_temperature_priority=None  IGBT_junction_temperature=25 degC  IGBT_junction_temperature_nominal_specify=off  IGBT_junction_temperature_nominal_value=1  IGBT_junction_temperature_nominal_unit=degC  diode_junction_temperature_specify=off  diode_junction_temperature_priority=None  diode_junction_temperature=25 degC  diode_junction_temperature_nominal_specify=off  diode_junction_temperature_nominal_value=1  diode_junction_temperature_nominal_unit=degC  Qj_specify=off  Qj_priority=None  Qj=0 W  Qj_nominal_specify=off  Qj_nominal_value=1  Qj_nominal_unit=W  accumulatedSwitchingLosses_specify=off  accumulatedSwitchingLosses_priority=None  accumulatedSwitchingLosses=0 J
  Simulink-PS Converter : nesl_utility/Simulink-PS Converter  PhysicalDomain=network_engine_domain  SubClassName=ps_input  LeftPortType=input  RightPortType=output  PseudoPeriodic=off  Frequencies=[]  NoiseDistribution=none  NoiseParameters=[]  Unit=V  AffineConversion=off  FilteringAndDerivatives=zero  SimscapeFilterOrder=1  InputFilterTimeConstant=.001  UdotUserProvided=1
  C : PMIOPort  Side=Right
  E : PMIOPort  Port=2  Side=Right
  wires:
  G/1 -> Simulink-PS Converter/1
  connections:
  Simulink-PS Converter/RConn1 -- IGBT/LConn1
  IGBT/RConn2 -- E/RConn1
  IGBT/RConn1 -- C/RConn1

== system MATE_SwitchedReluctanceMotor64Drive/Validation drive  only/Three-arm bridge/IGBT4 ==
  G : Inport
  IGBT : ee_lib/Semiconductors & Converters/IGBT (Ideal, Switching)  port_option=ee.enum.controlport.ps  Vf=0.1 V  Ron=0.01 Ohm  Goff=1e-5 1/Ohm  Vth=0.5 V  diode_param=ee.enum.semiconductors.protectionDiode.external  diode_Vf=0.6 V  diode_Ron=0.03 Ohm  diode_Goff=1e-5 1/Ohm  diode_C=5e-8 F  diode_iRM=-235 A  diode_iF=300 A  diode_idot=-50 A/us  diode_trr_param=1  diode_trr_factor=3  diode_trr=15 us  diode_Qrr=1.5e+3 s*uA  ice_specify=off  ice_priority=None  ice=0 A  ice_nominal_specify=off  ice_nominal_value=1  ice_nominal_unit=A  vce_specify=off  vce_priority=None  vce=0 V  vce_nominal_specify=off  vce_nominal_value=1  vce_nominal_unit=V  vge_specify=off  vge_priority=None  vge=0 V  vge_nominal_specify=off  vge_nominal_value=1  vge_nominal_unit=V  thermal_loss_option=ee.enum.converters.thermalLossOption.constantvalues  Von_data=[0, .1, .6, .8, 1, 1.3, 1.6, 2, 2.4; 0, .1, .7, 1, 1.2, 1.5, 1.9, 2.4, 2.8] V  Tj=[298.15, 398.15] K  Iout_data=[0, .1, 1, 5, 10, 20, 40, 70, 100] A  Eon_data=[0, .0024, .024, .12, .2, .48, 1.04, 2.16, 3.24; 0, .003, .03, .15, .25, .6, 1.3, 2.7, 4.05] * 1e-3 J  Eoff_data=[0, .0007, .0066, .033, .066, .17, .33, .83, 1.5; 0, .001, .01, .05, .1, .25, .5, 1.2, 2.2] * 1e-3 J  Eon_data_3D=[zeros(2, 9, 3)] J  Eoff_data_3D=[zeros(2, 9, 3)] J  Tj_loss=[298.15, 398.15] K  Iout_data_loss=[0, .1, 1, 5, 10, 20, 40, 70, 100] A  tabulateWithVce=false  Vce_loss=[0, 150, 300] V  Eon_scalar=22.86e-3 J  Eoff_scalar=17.14e-3 J  Voff=300 V  Iout_scalar=600 A  useCurrentFromPreviousCycle=false  useVoltageFromPreviousCycle=false  diodeModelType=ee.enum.converters.diodeModelType.pwl  diodeTableType=ee.enum.diode.tableType.IfMat  diode_ReverseIVType=ee.enum.diode.diodeReverseIV.constant  diode_IfMat=[.07, .12, .19, 1.75, 4.24, 7.32, 11.2; .16, .3, .72, 2.14, 4.02, 6.35, 9.12] A  diode_VfMat=[.9, 1.15, 1.25, 1.5, 1.75, 2.17, 2.6, 2.85; .58, .68, .75, 1.1, 1.38, 1.77, 2.27, 2.7] V  diode_TjVec=[25, 125] degC  diode_VfVec=[.5, .7, .9, 1.3, 1.7, 2.1, 2.5] V  diode_IfVec=[.1, .2, .5, 1, 2, 4, 7, 10] A  diode_IrMat=[1e-06, 2e-06, 5e-06, 1e-05, 2.5e-05, 5e-05, .0001; 2e-06, 5e-06, 1e-05, 4e-05, 8e-05, .0002, .0005] A  diode_VrMat=[10, 100, 200, 250, 300, 325, 350; 10, 70, 160, 220, 270, 300, 320] V  diode_VrVec=[10, 20, 40, 50, 70, 80, 100] V  diode_IrVec=[1e-06, 2e-06, 5e-06, 1e-05, 2e-05, 5e-05, .0001] A  diode_Vr=-600 V  diode_Ls=150 nH  diode_Erec=0.03 J  diode_rec_loss_model=ee.enum.diode.reverseRecoveryModel.fixed  diode_ErecVal=0 J  diode_scaleWithIandV=true  diode_ErecMat=zeros(2, 3) J  diode_TjrecVec=[298.15, 398.15] K  diode_IfrecVec=[.1, 1, 10] A  diode_IrecVal=10 A  diode_VrecVal=10 V  diode_tFilter=1 / 1000 / 100 s  separateThermalPortForDiode=false  thermal_network_parameterization=ee.enum.thermalNetworkTopology.external  Rth=[.08, .5] K/W  Rth_Cauer=[.08, .1, .5] K/W  Rth_Foster=[.08, .14, .22, .16] K/W  thermal_mass_parameterization=ee.enum.thermalNetwork.timeconstant  thermal_mass=[.01, .5] J/K  thermal_mass_Cauer=[.01, .1, .5] J/K  thermal_mass_Foster=[.001, .005, .05, .5] J/K  thermal_time_constant=[.001, .2] s  thermal_time_constant_Cauer=[.001, .1, .2] s  thermal_time_constant_Foster=[7e-05, .0007, .01, .08] s  thermal_mass_initial_temperatures=[25, 25] degC  thermal_mass_initial_temperatures_Cauer=[25, 25, 25] degC  junction_thermal_mass=0.01 J/K  Tvec_initial_Foster=[25, 25, 25, 25] degC  RthDiode=[.03, .2] K/W  RthCauerDiode=[.03, .1, .2] K/W  RthFosterDiode=[.03, .2] K/W  thermalMassDiode=[3, 25] J/K  thermalMassCauerDiode=[3, 10, 25] J/K  thermalMassFosterDiode=[33, 50] J/K  thermalTauDiode=[.1, 5] s  thermalTauCauerDiode=[.1, 1, 5] s  thermalTauFosterDiode=[1, 10] s  thermalMassInitTempDiode=[25, 25] degC  thermalMassInitTempCauerDiode=[25, 25, 25] degC  junctionthermalMassDiode=0.1 J/K  TVecInitialFosterDiode=[25, 25, 25, 25] degC  no_thermal_network=0  IGBT_junction_temperature_specify=off  IGBT_junction_temperature_priority=None  IGBT_junction_temperature=25 degC  IGBT_junction_temperature_nominal_specify=off  IGBT_junction_temperature_nominal_value=1  IGBT_junction_temperature_nominal_unit=degC  diode_junction_temperature_specify=off  diode_junction_temperature_priority=None  diode_junction_temperature=25 degC  diode_junction_temperature_nominal_specify=off  diode_junction_temperature_nominal_value=1  diode_junction_temperature_nominal_unit=degC  Qj_specify=off  Qj_priority=None  Qj=0 W  Qj_nominal_specify=off  Qj_nominal_value=1  Qj_nominal_unit=W  accumulatedSwitchingLosses_specify=off  accumulatedSwitchingLosses_priority=None  accumulatedSwitchingLosses=0 J
  Simulink-PS Converter : nesl_utility/Simulink-PS Converter  PhysicalDomain=network_engine_domain  SubClassName=ps_input  LeftPortType=input  RightPortType=output  PseudoPeriodic=off  Frequencies=[]  NoiseDistribution=none  NoiseParameters=[]  Unit=V  AffineConversion=off  FilteringAndDerivatives=zero  SimscapeFilterOrder=1  InputFilterTimeConstant=.001  UdotUserProvided=1
  C : PMIOPort  Side=Right
  E : PMIOPort  Port=2  Side=Right
  wires:
  G/1 -> Simulink-PS Converter/1
  connections:
  IGBT/RConn1 -- C/RConn1
  IGBT/RConn2 -- E/RConn1
  Simulink-PS Converter/RConn1 -- IGBT/LConn1
